simulink model "day05_compare_models"  (R2024a)
settings: Solver=ode45  StartTime=0.0  StopTime=6  RelTol=1e-8  AbsTol=1e-10
undefined symbols (not defined in the file or in its folder): m, t_step, U, v0, z0
settings Model: Creator=admin  LastModifiedBy=admin

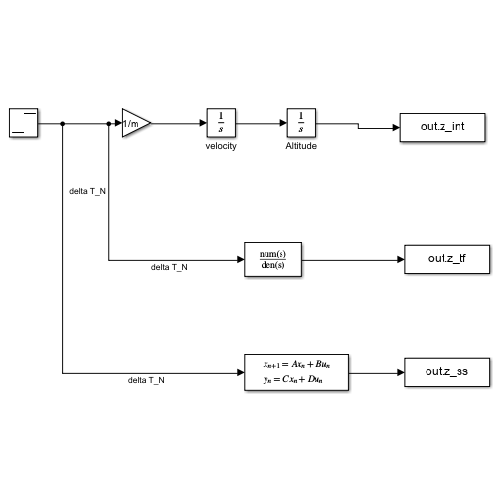
[thumbnail: Simulink's stored preview of the top-level diagram]
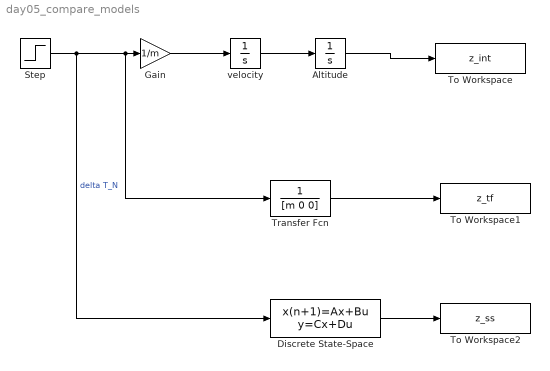
== system day05_compare_models ==
  Altitude : Integrator  InitialCondition=z0
  Discrete State-Space : DiscreteStateSpace  A=[0 1;0 0]  B=[0; 1/m]  C=[1 0]  D=0  InitialCondition=[z0; v0]  SampleTime=-1
  Gain : Gain  Gain=1/m
  Step : Step  Time=t_step  After=U  SampleTime=0
  To Workspace : ToWorkspace  VariableName=z_int  SaveFormat=Timeseries  SampleTime=-1
  To Workspace1 : ToWorkspace  VariableName=z_tf  SaveFormat=Timeseries  SampleTime=-1
  To Workspace2 : ToWorkspace  VariableName=z_ss  SaveFormat=Timeseries  SampleTime=-1
  Transfer Fcn : TransferFcn  Denominator=[m 0 0]
  velocity : Integrator  InitialCondition=v0
  wires:
  Gain/1 -> velocity/1
  velocity/1 -> Altitude/1
  Altitude/1 -> To Workspace/1
  Transfer Fcn/1 -> To Workspace1/1
  Discrete State-Space/1 -> To Workspace2/1
  Step/1 -> Discrete State-Space/1, Transfer Fcn/1, Gain/1  "delta T_N"
